simulink model "s_b16a4x1kf"  (R2018a)
settings: Solver=VariableStepDiscrete  StartTime=0.0  StopTime=1000  RelTol=1e-3
undefined symbols (not defined in the file): fft_stages, n_bits_ants, n_bits_xengs
libraries: xbsIndex_r4 x23740, casper_library_misc x48, casper_library_delays x8, xps_library x4, casper_library_scopes x1
(part 89 of 219)

== system s_b16a4x1kf/sys1/xeng/auto_tap/dual_pol_cmac ==
  a1 : Inport
  a2 : Inport  Port=2
  acc_in : Inport  Port=3
  sync : Inport  Port=4
  valid_in : Inport  Port=5
  Concat : xbsIndex_r4/Concat  num_inputs=4  dbl_ovrd=off  block_type=concat
      settings: block_version=9.2.01
  Constant1 : xbsIndex_r4/Constant  const=0  gui_display_data_type=Fixed-point  arith_type=Unsigned  n_bits=1  bin_pt=0  preci_type=Single  exp_width=8  frac_width=24  explicit_period=on  period=1  equ=P=C  opselect=C  inp2=PCIN>>17  opr=+  inp1=P  carry=CIN  dbl_ovrd=off  block_type=constant
      settings: block_version=9.2.01
  Constant2 : xbsIndex_r4/Constant  const=0  gui_display_data_type=Fixed-point  arith_type=Unsigned  n_bits=1  bin_pt=0  preci_type=Single  exp_width=8  frac_width=24  explicit_period=on  period=1  equ=P=C  opselect=C  inp2=PCIN>>17  opr=+  inp1=P  carry=CIN  dbl_ovrd=off  block_type=constant
      settings: block_version=9.2.01
  Constant4 : xbsIndex_r4/Constant  const=0  gui_display_data_type=Fixed-point  arith_type=Unsigned  n_bits=1  bin_pt=0  preci_type=Single  exp_width=8  frac_width=24  explicit_period=on  period=1  equ=P=C  opselect=C  inp2=PCIN>>17  opr=+  inp1=P  carry=CIN  dbl_ovrd=off  block_type=constant
      settings: block_version=9.2.01
  Slice{,1,6,10} (4 alike) : xbsIndex_r4/Slice  nbits=2*n_bits_in  boolean_output=off  mode=Upper Bit Location + Width  bit1=0  base1=MSB of Input  bit0=0  base0=LSB of Input  dbl_ovrd=off  block_type=slice
      settings: block_version=9.2.01
  Slice11 : xbsIndex_r4/Slice  nbits=2*n_bits_out  boolean_output=off  mode=Upper Bit Location + Width  bit1=-6*n_bits_out  base1=MSB of Input  bit0=0  base0=LSB of Input  dbl_ovrd=off  block_type=slice
      settings: infoedit="Extracts a given range of bits from each input sample and presents it at the output.  The output type is ordinarily unsigned with binary point at zero, but can be Boolean when the slice is one bit wide.<P><P>Hardware notes: In hardware this block costs nothing."  block_version=9.2.01
  Slice2 : xbsIndex_r4/Slice  nbits=2*n_bits_out  boolean_output=off  mode=Upper Bit Location + Width  bit1=0  base1=MSB of Input  bit0=0  base0=LSB of Input  dbl_ovrd=off  block_type=slice
      settings: infoedit="Extracts a given range of bits from each input sample and presents it at the output.  The output type is ordinarily unsigned with binary point at zero, but can be Boolean when the slice is one bit wide.<P><P>Hardware notes: In hardware this block costs nothing."  block_version=9.2.01
  Slice{3..4,7,9} (4 alike) : xbsIndex_r4/Slice  nbits=2*n_bits_in  boolean_output=off  mode=Upper Bit Location + Width  bit1=-2*n_bits_in  base1=MSB of Input  bit0=0  base0=LSB of Input  dbl_ovrd=off  block_type=slice
      settings: block_version=9.2.01
  Slice5 : xbsIndex_r4/Slice  nbits=2*n_bits_out  boolean_output=off  mode=Upper Bit Location + Width  bit1=-2*n_bits_out  base1=MSB of Input  bit0=0  base0=LSB of Input  dbl_ovrd=off  block_type=slice
      settings: infoedit="Extracts a given range of bits from each input sample and presents it at the output.  The output type is ordinarily unsigned with binary point at zero, but can be Boolean when the slice is one bit wide.<P><P>Hardware notes: In hardware this block costs nothing."  block_version=9.2.01
  Slice8 : xbsIndex_r4/Slice  nbits=2*n_bits_out  boolean_output=off  mode=Upper Bit Location + Width  bit1=-4*n_bits_out  base1=MSB of Input  bit0=0  base0=LSB of Input  dbl_ovrd=off  block_type=slice
      settings: infoedit="Extracts a given range of bits from each input sample and presents it at the output.  The output type is ordinarily unsigned with binary point at zero, but can be Boolean when the slice is one bit wide.<P><P>Hardware notes: In hardware this block costs nothing."  block_version=9.2.01
  Terminator : Terminator
  Terminator1 : Terminator
  Terminator2 : Terminator
  cmac : Subsystem  Tag=cmac  AncestorBlock=casper_library_correlator/cmac  mask(cmac){acc_len=256, n_bits_a=8, bin_pt_a=7, n_bits_b=8, bin_pt_b=7, quantization=Truncate, overflow=Wrap, mult_latency=4, add_latency=3, in_latency=0, conv_latency=0, multiplier_implementation=embedded multiplier core}
      mask prompts: acc_len "Number of Accumulations"; n_bits_a "Number of bits 'a'"; bin_pt_a "Binary point 'a'"; n_bits_b "Number of bits 'b'"; bin_pt_b "Binary point 'b'"; quantization "Quantisation"; mult_latency "Multiplier Latency"; add_latency "Adder Latency"; in_latency "Input Latency"; conv_latency "Convert Latency"; multiplier_implementation "Multiplier Implementation"
      mask help: A complex multiply-accumulate block. Full precision.
      mask init: same as s_b16a4x1kf/sys0/xeng/auto_tap/dual_pol_cmac/cmac
      mask TypeOptions quantization: Truncate | Round  (unbiased: +/- Inf) | Round  (unbiased: Even Values)
      mask TypeOptions overflow: Wrap | Saturate | Flag as error
      mask TypeOptions multiplier_implementation: behavioral HDL | standard core | embedded multiplier core
  cmac1 : Subsystem  Tag=cmac  AncestorBlock=casper_library_correlator/cmac  mask(cmac){acc_len=256, n_bits_a=8, bin_pt_a=7, n_bits_b=8, bin_pt_b=7, quantization=Truncate, overflow=Wrap, mult_latency=4, add_latency=3, in_latency=0, conv_latency=0, multiplier_implementation=embedded multiplier core}
      mask prompts: acc_len "Number of Accumulations"; n_bits_a "Number of bits 'a'"; bin_pt_a "Binary point 'a'"; n_bits_b "Number of bits 'b'"; bin_pt_b "Binary point 'b'"; quantization "Quantisation"; mult_latency "Multiplier Latency"; add_latency "Adder Latency"; in_latency "Input Latency"; conv_latency "Convert Latency"; multiplier_implementation "Multiplier Implementation"
      mask help: A complex multiply-accumulate block. Full precision.
      mask init: same as s_b16a4x1kf/sys0/xeng/auto_tap/dual_pol_cmac/cmac
      mask TypeOptions quantization: Truncate | Round  (unbiased: +/- Inf) | Round  (unbiased: Even Values)
      mask TypeOptions overflow: Wrap | Saturate | Flag as error
      mask TypeOptions multiplier_implementation: behavioral HDL | standard core | embedded multiplier core
  cmac2 : Subsystem  Tag=cmac  AncestorBlock=casper_library_correlator/cmac  mask(cmac){acc_len=256, n_bits_a=8, bin_pt_a=7, n_bits_b=8, bin_pt_b=7, quantization=Truncate, overflow=Wrap, mult_latency=4, add_latency=3, in_latency=0, conv_latency=0, multiplier_implementation=embedded multiplier core}
      mask prompts: acc_len "Number of Accumulations"; n_bits_a "Number of bits 'a'"; bin_pt_a "Binary point 'a'"; n_bits_b "Number of bits 'b'"; bin_pt_b "Binary point 'b'"; quantization "Quantisation"; mult_latency "Multiplier Latency"; add_latency "Adder Latency"; in_latency "Input Latency"; conv_latency "Convert Latency"; multiplier_implementation "Multiplier Implementation"
      mask help: A complex multiply-accumulate block. Full precision.
      mask init: same as s_b16a4x1kf/sys0/xeng/auto_tap/dual_pol_cmac/cmac
      mask TypeOptions quantization: Truncate | Round  (unbiased: +/- Inf) | Round  (unbiased: Even Values)
      mask TypeOptions overflow: Wrap | Saturate | Flag as error
      mask TypeOptions multiplier_implementation: behavioral HDL | standard core | embedded multiplier core
  cmac3 : Subsystem  Tag=cmac  AncestorBlock=casper_library_correlator/cmac  mask(cmac){acc_len=256, n_bits_a=8, bin_pt_a=7, n_bits_b=8, bin_pt_b=7, quantization=Truncate, overflow=Wrap, mult_latency=4, add_latency=3, in_latency=0, conv_latency=0, multiplier_implementation=embedded multiplier core}
      mask prompts: acc_len "Number of Accumulations"; n_bits_a "Number of bits 'a'"; bin_pt_a "Binary point 'a'"; n_bits_b "Number of bits 'b'"; bin_pt_b "Binary point 'b'"; quantization "Quantisation"; mult_latency "Multiplier Latency"; add_latency "Adder Latency"; in_latency "Input Latency"; conv_latency "Convert Latency"; multiplier_implementation "Multiplier Implementation"
      mask help: A complex multiply-accumulate block. Full precision.
      mask init: same as s_b16a4x1kf/sys0/xeng/auto_tap/dual_pol_cmac/cmac
      mask TypeOptions quantization: Truncate | Round  (unbiased: +/- Inf) | Round  (unbiased: Even Values)
      mask TypeOptions overflow: Wrap | Saturate | Flag as error
      mask TypeOptions multiplier_implementation: behavioral HDL | standard core | embedded multiplier core
  acc_out : Outport
  valid_out : Outport  Port=2
  wires:
  Constant2/1 -> cmac/5(valid_in)
  Slice/1 -> cmac/1(a+bi)
  Slice1/1 -> cmac/2(c+di)
  Slice2/1 -> cmac/3(acc_in)
  Slice3/1 -> cmac1/1(a+bi)
  Slice4/1 -> cmac1/2(c+di)
  Slice5/1 -> cmac1/3(acc_in)
  Concat/1 -> acc_out/1
  valid_in/1 -> cmac3/5(valid_in)
  cmac/2(valid_out) -> Terminator/1
  Constant1/1 -> cmac1/5(valid_in)
  Slice6/1 -> cmac2/1(a+bi)
  Slice7/1 -> cmac2/2(c+di)
  Slice8/1 -> cmac2/3(acc_in)
  Constant4/1 -> cmac2/5(valid_in)
  Slice9/1 -> cmac3/1(a+bi)
  Slice10/1 -> cmac3/2(c+di)
  Slice11/1 -> cmac3/3(acc_in)
  sync/1 -> cmac/4(sync), cmac1/4(sync), cmac2/4(sync), cmac3/4(sync)
  cmac1/2(valid_out) -> Terminator1/1
  cmac2/2(valid_out) -> Terminator2/1
  cmac3/2(valid_out) -> valid_out/1
  cmac/1(acc_out) -> Concat/1
  cmac1/1(acc_out) -> Concat/2
  cmac2/1(acc_out) -> Concat/3
  cmac3/1(acc_out) -> Concat/4
  a1/1 -> Slice/1, Slice3/1, Slice6/1, Slice9/1
  a2/1 -> Slice1/1, Slice4/1, Slice7/1, Slice10/1
  acc_in/1 -> Slice11/1, Slice8/1, Slice5/1, Slice2/1

== system s_b16a4x1kf/sys1/xeng/baseline_tap1/delay ==
  din : Inport
  constant : xbsIndex_r4/Constant  const=1  gui_display_data_type=Fixed-point  arith_type=Boolean  n_bits=16  bin_pt=14  preci_type=Single  exp_width=8  frac_width=24  explicit_period=on  period=1  equ=P=C  opselect=C  inp2=PCIN>>17  opr=+  inp1=P  carry=CIN  dbl_ovrd=off  block_type=constant
  counter : xbsIndex_r4/Counter  cnt_type=Count Limited  cnt_to=DelayLen - bram_latency - 1  operation=Up  start_count=0  cnt_by_val=1  arith_type=Unsigned  n_bits=8  bin_pt=0  load_pin=off  rst=off  en=off  explicit_period=on  period=1  use_behavioral_HDL=on  implementation=Fabric  use_rpm=off  dbl_ovrd=off  block_type=counter
  d{1..6} (6 alike) : xbsIndex_r4/Delay  rst=off  infoeditControl=Selection of Reset will increase slice count due to use of real FFs and instead of SRLs  en=off  latency=1  reg_retiming=on  dbl_ovrd=off  block_type=delay
  ram : xbsIndex_r4/Single Port RAM  depth=256  initVector=0  distributed_mem=Block RAM  write_mode=Read Before Write  rst=off  init_reg=0  en=off  latency=1  optimize=Area  dbl_ovrd=off  block_type=spram
  dout : Outport
  wires:
  counter/1 -> ram/1
  din/1 -> ram/2
  constant/1 -> ram/3
  ram/1 -> d1/1
  d1/1 -> d2/1
  d2/1 -> d3/1
  d3/1 -> d4/1
  d4/1 -> d5/1
  d5/1 -> d6/1
  d6/1 -> dout/1

== system s_b16a4x1kf/sys1/xeng/baseline_tap1/dual_pol_cmac ==
  a1 : Inport
  a2 : Inport  Port=2
  acc_in : Inport  Port=3
  sync : Inport  Port=4
  valid_in : Inport  Port=5
  Concat : xbsIndex_r4/Concat  num_inputs=4  dbl_ovrd=off  block_type=concat
      settings: block_version=9.2.01
  Constant1 : xbsIndex_r4/Constant  const=0  gui_display_data_type=Fixed-point  arith_type=Unsigned  n_bits=1  bin_pt=0  preci_type=Single  exp_width=8  frac_width=24  explicit_period=on  period=1  equ=P=C  opselect=C  inp2=PCIN>>17  opr=+  inp1=P  carry=CIN  dbl_ovrd=off  block_type=constant
      settings: block_version=9.2.01
  Constant2 : xbsIndex_r4/Constant  const=0  gui_display_data_type=Fixed-point  arith_type=Unsigned  n_bits=1  bin_pt=0  preci_type=Single  exp_width=8  frac_width=24  explicit_period=on  period=1  equ=P=C  opselect=C  inp2=PCIN>>17  opr=+  inp1=P  carry=CIN  dbl_ovrd=off  block_type=constant
      settings: block_version=9.2.01
  Constant4 : xbsIndex_r4/Constant  const=0  gui_display_data_type=Fixed-point  arith_type=Unsigned  n_bits=1  bin_pt=0  preci_type=Single  exp_width=8  frac_width=24  explicit_period=on  period=1  equ=P=C  opselect=C  inp2=PCIN>>17  opr=+  inp1=P  carry=CIN  dbl_ovrd=off  block_type=constant
      settings: block_version=9.2.01
  Slice{,1,6,10} (4 alike) : xbsIndex_r4/Slice  nbits=2*n_bits_in  boolean_output=off  mode=Upper Bit Location + Width  bit1=0  base1=MSB of Input  bit0=0  base0=LSB of Input  dbl_ovrd=off  block_type=slice
      settings: block_version=9.2.01
  Slice11 : xbsIndex_r4/Slice  nbits=2*n_bits_out  boolean_output=off  mode=Upper Bit Location + Width  bit1=-6*n_bits_out  base1=MSB of Input  bit0=0  base0=LSB of Input  dbl_ovrd=off  block_type=slice
      settings: infoedit="Extracts a given range of bits from each input sample and presents it at the output.  The output type is ordinarily unsigned with binary point at zero, but can be Boolean when the slice is one bit wide.<P><P>Hardware notes: In hardware this block costs nothing."  block_version=9.2.01
  Slice2 : xbsIndex_r4/Slice  nbits=2*n_bits_out  boolean_output=off  mode=Upper Bit Location + Width  bit1=0  base1=MSB of Input  bit0=0  base0=LSB of Input  dbl_ovrd=off  block_type=slice
      settings: infoedit="Extracts a given range of bits from each input sample and presents it at the output.  The output type is ordinarily unsigned with binary point at zero, but can be Boolean when the slice is one bit wide.<P><P>Hardware notes: In hardware this block costs nothing."  block_version=9.2.01
  Slice{3..4,7,9} (4 alike) : xbsIndex_r4/Slice  nbits=2*n_bits_in  boolean_output=off  mode=Upper Bit Location + Width  bit1=-2*n_bits_in  base1=MSB of Input  bit0=0  base0=LSB of Input  dbl_ovrd=off  block_type=slice
      settings: block_version=9.2.01
  Slice5 : xbsIndex_r4/Slice  nbits=2*n_bits_out  boolean_output=off  mode=Upper Bit Location + Width  bit1=-2*n_bits_out  base1=MSB of Input  bit0=0  base0=LSB of Input  dbl_ovrd=off  block_type=slice
      settings: infoedit="Extracts a given range of bits from each input sample and presents it at the output.  The output type is ordinarily unsigned with binary point at zero, but can be Boolean when the slice is one bit wide.<P><P>Hardware notes: In hardware this block costs nothing."  block_version=9.2.01
  Slice8 : xbsIndex_r4/Slice  nbits=2*n_bits_out  boolean_output=off  mode=Upper Bit Location + Width  bit1=-4*n_bits_out  base1=MSB of Input  bit0=0  base0=LSB of Input  dbl_ovrd=off  block_type=slice
      settings: infoedit="Extracts a given range of bits from each input sample and presents it at the output.  The output type is ordinarily unsigned with binary point at zero, but can be Boolean when the slice is one bit wide.<P><P>Hardware notes: In hardware this block costs nothing."  block_version=9.2.01
  Terminator : Terminator
  Terminator1 : Terminator
  Terminator2 : Terminator
  cmac : Subsystem  Tag=cmac  AncestorBlock=casper_library_correlator/cmac  mask(cmac){acc_len=256, n_bits_a=8, bin_pt_a=7, n_bits_b=8, bin_pt_b=7, quantization=Truncate, overflow=Wrap, mult_latency=4, add_latency=3, in_latency=0, conv_latency=0, multiplier_implementation=embedded multiplier core}
      mask prompts: acc_len "Number of Accumulations"; n_bits_a "Number of bits 'a'"; bin_pt_a "Binary point 'a'"; n_bits_b "Number of bits 'b'"; bin_pt_b "Binary point 'b'"; quantization "Quantisation"; mult_latency "Multiplier Latency"; add_latency "Adder Latency"; in_latency "Input Latency"; conv_latency "Convert Latency"; multiplier_implementation "Multiplier Implementation"
      mask help: A complex multiply-accumulate block. Full precision.
      mask init: same as s_b16a4x1kf/sys0/xeng/auto_tap/dual_pol_cmac/cmac
      mask TypeOptions quantization: Truncate | Round  (unbiased: +/- Inf) | Round  (unbiased: Even Values)
      mask TypeOptions overflow: Wrap | Saturate | Flag as error
      mask TypeOptions multiplier_implementation: behavioral HDL | standard core | embedded multiplier core
  cmac1 : Subsystem  Tag=cmac  AncestorBlock=casper_library_correlator/cmac  mask(cmac){acc_len=256, n_bits_a=8, bin_pt_a=7, n_bits_b=8, bin_pt_b=7, quantization=Truncate, overflow=Wrap, mult_latency=4, add_latency=3, in_latency=0, conv_latency=0, multiplier_implementation=embedded multiplier core}
      mask prompts: acc_len "Number of Accumulations"; n_bits_a "Number of bits 'a'"; bin_pt_a "Binary point 'a'"; n_bits_b "Number of bits 'b'"; bin_pt_b "Binary point 'b'"; quantization "Quantisation"; mult_latency "Multiplier Latency"; add_latency "Adder Latency"; in_latency "Input Latency"; conv_latency "Convert Latency"; multiplier_implementation "Multiplier Implementation"
      mask help: A complex multiply-accumulate block. Full precision.
      mask init: same as s_b16a4x1kf/sys0/xeng/auto_tap/dual_pol_cmac/cmac
      mask TypeOptions quantization: Truncate | Round  (unbiased: +/- Inf) | Round  (unbiased: Even Values)
      mask TypeOptions overflow: Wrap | Saturate | Flag as error
      mask TypeOptions multiplier_implementation: behavioral HDL | standard core | embedded multiplier core
  cmac2 : Subsystem  Tag=cmac  AncestorBlock=casper_library_correlator/cmac  mask(cmac){acc_len=256, n_bits_a=8, bin_pt_a=7, n_bits_b=8, bin_pt_b=7, quantization=Truncate, overflow=Wrap, mult_latency=4, add_latency=3, in_latency=0, conv_latency=0, multiplier_implementation=embedded multiplier core}
      mask prompts: acc_len "Number of Accumulations"; n_bits_a "Number of bits 'a'"; bin_pt_a "Binary point 'a'"; n_bits_b "Number of bits 'b'"; bin_pt_b "Binary point 'b'"; quantization "Quantisation"; mult_latency "Multiplier Latency"; add_latency "Adder Latency"; in_latency "Input Latency"; conv_latency "Convert Latency"; multiplier_implementation "Multiplier Implementation"
      mask help: A complex multiply-accumulate block. Full precision.
      mask init: same as s_b16a4x1kf/sys0/xeng/auto_tap/dual_pol_cmac/cmac
      mask TypeOptions quantization: Truncate | Round  (unbiased: +/- Inf) | Round  (unbiased: Even Values)
      mask TypeOptions overflow: Wrap | Saturate | Flag as error
      mask TypeOptions multiplier_implementation: behavioral HDL | standard core | embedded multiplier core
  cmac3 : Subsystem  Tag=cmac  AncestorBlock=casper_library_correlator/cmac  mask(cmac){acc_len=256, n_bits_a=8, bin_pt_a=7, n_bits_b=8, bin_pt_b=7, quantization=Truncate, overflow=Wrap, mult_latency=4, add_latency=3, in_latency=0, conv_latency=0, multiplier_implementation=embedded multiplier core}
      mask prompts: acc_len "Number of Accumulations"; n_bits_a "Number of bits 'a'"; bin_pt_a "Binary point 'a'"; n_bits_b "Number of bits 'b'"; bin_pt_b "Binary point 'b'"; quantization "Quantisation"; mult_latency "Multiplier Latency"; add_latency "Adder Latency"; in_latency "Input Latency"; conv_latency "Convert Latency"; multiplier_implementation "Multiplier Implementation"
      mask help: A complex multiply-accumulate block. Full precision.
      mask init: same as s_b16a4x1kf/sys0/xeng/auto_tap/dual_pol_cmac/cmac
      mask TypeOptions quantization: Truncate | Round  (unbiased: +/- Inf) | Round  (unbiased: Even Values)
      mask TypeOptions overflow: Wrap | Saturate | Flag as error
      mask TypeOptions multiplier_implementation: behavioral HDL | standard core | embedded multiplier core
  acc_out : Outport
  valid_out : Outport  Port=2
  wires:
  Constant2/1 -> cmac/5(valid_in)
  Slice/1 -> cmac/1(a+bi)
  Slice1/1 -> cmac/2(c+di)
  Slice2/1 -> cmac/3(acc_in)
  Slice3/1 -> cmac1/1(a+bi)
  Slice4/1 -> cmac1/2(c+di)
  Slice5/1 -> cmac1/3(acc_in)
  Concat/1 -> acc_out/1
  valid_in/1 -> cmac3/5(valid_in)
  cmac/2(valid_out) -> Terminator/1
  Constant1/1 -> cmac1/5(valid_in)
  Slice6/1 -> cmac2/1(a+bi)
  Slice7/1 -> cmac2/2(c+di)
  Slice8/1 -> cmac2/3(acc_in)
  Constant4/1 -> cmac2/5(valid_in)
  Slice9/1 -> cmac3/1(a+bi)
  Slice10/1 -> cmac3/2(c+di)
  Slice11/1 -> cmac3/3(acc_in)
  sync/1 -> cmac/4(sync), cmac1/4(sync), cmac2/4(sync), cmac3/4(sync)
  cmac1/2(valid_out) -> Terminator1/1
  cmac2/2(valid_out) -> Terminator2/1
  cmac3/2(valid_out) -> valid_out/1
  cmac/1(acc_out) -> Concat/1
  cmac1/1(acc_out) -> Concat/2
  cmac2/1(acc_out) -> Concat/3
  cmac3/1(acc_out) -> Concat/4
  a1/1 -> Slice/1, Slice3/1, Slice6/1, Slice9/1
  a2/1 -> Slice1/1, Slice4/1, Slice7/1, Slice10/1
  acc_in/1 -> Slice11/1, Slice8/1, Slice5/1, Slice2/1

== system s_b16a4x1kf/sys1/xeng/baseline_tap2/delay ==
  din : Inport
  constant : xbsIndex_r4/Constant  const=1  gui_display_data_type=Fixed-point  arith_type=Boolean  n_bits=16  bin_pt=14  preci_type=Single  exp_width=8  frac_width=24  explicit_period=on  period=1  equ=P=C  opselect=C  inp2=PCIN>>17  opr=+  inp1=P  carry=CIN  dbl_ovrd=off  block_type=constant
  counter : xbsIndex_r4/Counter  cnt_type=Count Limited  cnt_to=DelayLen - bram_latency - 1  operation=Up  start_count=0  cnt_by_val=1  arith_type=Unsigned  n_bits=8  bin_pt=0  load_pin=off  rst=off  en=off  explicit_period=on  period=1  use_behavioral_HDL=on  implementation=Fabric  use_rpm=off  dbl_ovrd=off  block_type=counter
  d{1..6} (6 alike) : xbsIndex_r4/Delay  rst=off  infoeditControl=Selection of Reset will increase slice count due to use of real FFs and instead of SRLs  en=off  latency=1  reg_retiming=on  dbl_ovrd=off  block_type=delay
  ram : xbsIndex_r4/Single Port RAM  depth=256  initVector=0  distributed_mem=Block RAM  write_mode=Read Before Write  rst=off  init_reg=0  en=off  latency=1  optimize=Area  dbl_ovrd=off  block_type=spram
  dout : Outport
  wires:
  counter/1 -> ram/1
  din/1 -> ram/2
  constant/1 -> ram/3
  ram/1 -> d1/1
  d1/1 -> d2/1
  d2/1 -> d3/1
  d3/1 -> d4/1
  d4/1 -> d5/1
  d5/1 -> d6/1
  d6/1 -> dout/1

== system s_b16a4x1kf/sys1/xeng/baseline_tap2/dual_pol_cmac ==
  a1 : Inport
  a2 : Inport  Port=2
  acc_in : Inport  Port=3
  sync : Inport  Port=4
  valid_in : Inport  Port=5
  Concat : xbsIndex_r4/Concat  num_inputs=4  dbl_ovrd=off  block_type=concat
      settings: block_version=9.2.01
  Constant1 : xbsIndex_r4/Constant  const=0  gui_display_data_type=Fixed-point  arith_type=Unsigned  n_bits=1  bin_pt=0  preci_type=Single  exp_width=8  frac_width=24  explicit_period=on  period=1  equ=P=C  opselect=C  inp2=PCIN>>17  opr=+  inp1=P  carry=CIN  dbl_ovrd=off  block_type=constant
      settings: block_version=9.2.01
  Constant2 : xbsIndex_r4/Constant  const=0  gui_display_data_type=Fixed-point  arith_type=Unsigned  n_bits=1  bin_pt=0  preci_type=Single  exp_width=8  frac_width=24  explicit_period=on  period=1  equ=P=C  opselect=C  inp2=PCIN>>17  opr=+  inp1=P  carry=CIN  dbl_ovrd=off  block_type=constant
      settings: block_version=9.2.01
  Constant4 : xbsIndex_r4/Constant  const=0  gui_display_data_type=Fixed-point  arith_type=Unsigned  n_bits=1  bin_pt=0  preci_type=Single  exp_width=8  frac_width=24  explicit_period=on  period=1  equ=P=C  opselect=C  inp2=PCIN>>17  opr=+  inp1=P  carry=CIN  dbl_ovrd=off  block_type=constant
      settings: block_version=9.2.01
  Slice{,1,6,10} (4 alike) : xbsIndex_r4/Slice  nbits=2*n_bits_in  boolean_output=off  mode=Upper Bit Location + Width  bit1=0  base1=MSB of Input  bit0=0  base0=LSB of Input  dbl_ovrd=off  block_type=slice
      settings: block_version=9.2.01
  Slice11 : xbsIndex_r4/Slice  nbits=2*n_bits_out  boolean_output=off  mode=Upper Bit Location + Width  bit1=-6*n_bits_out  base1=MSB of Input  bit0=0  base0=LSB of Input  dbl_ovrd=off  block_type=slice
      settings: infoedit="Extracts a given range of bits from each input sample and presents it at the output.  The output type is ordinarily unsigned with binary point at zero, but can be Boolean when the slice is one bit wide.<P><P>Hardware notes: In hardware this block costs nothing."  block_version=9.2.01
  Slice2 : xbsIndex_r4/Slice  nbits=2*n_bits_out  boolean_output=off  mode=Upper Bit Location + Width  bit1=0  base1=MSB of Input  bit0=0  base0=LSB of Input  dbl_ovrd=off  block_type=slice
      settings: infoedit="Extracts a given range of bits from each input sample and presents it at the output.  The output type is ordinarily unsigned with binary point at zero, but can be Boolean when the slice is one bit wide.<P><P>Hardware notes: In hardware this block costs nothing."  block_version=9.2.01
  Slice{3..4,7,9} (4 alike) : xbsIndex_r4/Slice  nbits=2*n_bits_in  boolean_output=off  mode=Upper Bit Location + Width  bit1=-2*n_bits_in  base1=MSB of Input  bit0=0  base0=LSB of Input  dbl_ovrd=off  block_type=slice
      settings: block_version=9.2.01
  Slice5 : xbsIndex_r4/Slice  nbits=2*n_bits_out  boolean_output=off  mode=Upper Bit Location + Width  bit1=-2*n_bits_out  base1=MSB of Input  bit0=0  base0=LSB of Input  dbl_ovrd=off  block_type=slice
      settings: infoedit="Extracts a given range of bits from each input sample and presents it at the output.  The output type is ordinarily unsigned with binary point at zero, but can be Boolean when the slice is one bit wide.<P><P>Hardware notes: In hardware this block costs nothing."  block_version=9.2.01
  Slice8 : xbsIndex_r4/Slice  nbits=2*n_bits_out  boolean_output=off  mode=Upper Bit Location + Width  bit1=-4*n_bits_out  base1=MSB of Input  bit0=0  base0=LSB of Input  dbl_ovrd=off  block_type=slice
      settings: infoedit="Extracts a given range of bits from each input sample and presents it at the output.  The output type is ordinarily unsigned with binary point at zero, but can be Boolean when the slice is one bit wide.<P><P>Hardware notes: In hardware this block costs nothing."  block_version=9.2.01
  Terminator : Terminator
  Terminator1 : Terminator
  Terminator2 : Terminator
  cmac : Subsystem  Tag=cmac  AncestorBlock=casper_library_correlator/cmac  mask(cmac){acc_len=256, n_bits_a=8, bin_pt_a=7, n_bits_b=8, bin_pt_b=7, quantization=Truncate, overflow=Wrap, mult_latency=4, add_latency=3, in_latency=0, conv_latency=0, multiplier_implementation=embedded multiplier core}
      mask prompts: acc_len "Number of Accumulations"; n_bits_a "Number of bits 'a'"; bin_pt_a "Binary point 'a'"; n_bits_b "Number of bits 'b'"; bin_pt_b "Binary point 'b'"; quantization "Quantisation"; mult_latency "Multiplier Latency"; add_latency "Adder Latency"; in_latency "Input Latency"; conv_latency "Convert Latency"; multiplier_implementation "Multiplier Implementation"
      mask help: A complex multiply-accumulate block. Full precision.
      mask init: same as s_b16a4x1kf/sys0/xeng/auto_tap/dual_pol_cmac/cmac
      mask TypeOptions quantization: Truncate | Round  (unbiased: +/- Inf) | Round  (unbiased: Even Values)
      mask TypeOptions overflow: Wrap | Saturate | Flag as error
      mask TypeOptions multiplier_implementation: behavioral HDL | standard core | embedded multiplier core
  cmac1 : Subsystem  Tag=cmac  AncestorBlock=casper_library_correlator/cmac  mask(cmac){acc_len=256, n_bits_a=8, bin_pt_a=7, n_bits_b=8, bin_pt_b=7, quantization=Truncate, overflow=Wrap, mult_latency=4, add_latency=3, in_latency=0, conv_latency=0, multiplier_implementation=embedded multiplier core}
      mask prompts: acc_len "Number of Accumulations"; n_bits_a "Number of bits 'a'"; bin_pt_a "Binary point 'a'"; n_bits_b "Number of bits 'b'"; bin_pt_b "Binary point 'b'"; quantization "Quantisation"; mult_latency "Multiplier Latency"; add_latency "Adder Latency"; in_latency "Input Latency"; conv_latency "Convert Latency"; multiplier_implementation "Multiplier Implementation"
      mask help: A complex multiply-accumulate block. Full precision.
      mask init: same as s_b16a4x1kf/sys0/xeng/auto_tap/dual_pol_cmac/cmac
      mask TypeOptions quantization: Truncate | Round  (unbiased: +/- Inf) | Round  (unbiased: Even Values)
      mask TypeOptions overflow: Wrap | Saturate | Flag as error
      mask TypeOptions multiplier_implementation: behavioral HDL | standard core | embedded multiplier core
  cmac2 : Subsystem  Tag=cmac  AncestorBlock=casper_library_correlator/cmac  mask(cmac){acc_len=256, n_bits_a=8, bin_pt_a=7, n_bits_b=8, bin_pt_b=7, quantization=Truncate, overflow=Wrap, mult_latency=4, add_latency=3, in_latency=0, conv_latency=0, multiplier_implementation=embedded multiplier core}
      mask prompts: acc_len "Number of Accumulations"; n_bits_a "Number of bits 'a'"; bin_pt_a "Binary point 'a'"; n_bits_b "Number of bits 'b'"; bin_pt_b "Binary point 'b'"; quantization "Quantisation"; mult_latency "Multiplier Latency"; add_latency "Adder Latency"; in_latency "Input Latency"; conv_latency "Convert Latency"; multiplier_implementation "Multiplier Implementation"
      mask help: A complex multiply-accumulate block. Full precision.
      mask init: same as s_b16a4x1kf/sys0/xeng/auto_tap/dual_pol_cmac/cmac
      mask TypeOptions quantization: Truncate | Round  (unbiased: +/- Inf) | Round  (unbiased: Even Values)
      mask TypeOptions overflow: Wrap | Saturate | Flag as error
      mask TypeOptions multiplier_implementation: behavioral HDL | standard core | embedded multiplier core
  cmac3 : Subsystem  Tag=cmac  AncestorBlock=casper_library_correlator/cmac  mask(cmac){acc_len=256, n_bits_a=8, bin_pt_a=7, n_bits_b=8, bin_pt_b=7, quantization=Truncate, overflow=Wrap, mult_latency=4, add_latency=3, in_latency=0, conv_latency=0, multiplier_implementation=embedded multiplier core}
      mask prompts: acc_len "Number of Accumulations"; n_bits_a "Number of bits 'a'"; bin_pt_a "Binary point 'a'"; n_bits_b "Number of bits 'b'"; bin_pt_b "Binary point 'b'"; quantization "Quantisation"; mult_latency "Multiplier Latency"; add_latency "Adder Latency"; in_latency "Input Latency"; conv_latency "Convert Latency"; multiplier_implementation "Multiplier Implementation"
      mask help: A complex multiply-accumulate block. Full precision.
      mask init: same as s_b16a4x1kf/sys0/xeng/auto_tap/dual_pol_cmac/cmac
      mask TypeOptions quantization: Truncate | Round  (unbiased: +/- Inf) | Round  (unbiased: Even Values)
      mask TypeOptions overflow: Wrap | Saturate | Flag as error
      mask TypeOptions multiplier_implementation: behavioral HDL | standard core | embedded multiplier core
  acc_out : Outport
  valid_out : Outport  Port=2
  wires:
  Constant2/1 -> cmac/5(valid_in)
  Slice/1 -> cmac/1(a+bi)
  Slice1/1 -> cmac/2(c+di)
  Slice2/1 -> cmac/3(acc_in)
  Slice3/1 -> cmac1/1(a+bi)
  Slice4/1 -> cmac1/2(c+di)
  Slice5/1 -> cmac1/3(acc_in)
  Concat/1 -> acc_out/1
  valid_in/1 -> cmac3/5(valid_in)
  cmac/2(valid_out) -> Terminator/1
  Constant1/1 -> cmac1/5(valid_in)
  Slice6/1 -> cmac2/1(a+bi)
  Slice7/1 -> cmac2/2(c+di)
  Slice8/1 -> cmac2/3(acc_in)
  Constant4/1 -> cmac2/5(valid_in)
  Slice9/1 -> cmac3/1(a+bi)
  Slice10/1 -> cmac3/2(c+di)
  Slice11/1 -> cmac3/3(acc_in)
  sync/1 -> cmac/4(sync), cmac1/4(sync), cmac2/4(sync), cmac3/4(sync)
  cmac1/2(valid_out) -> Terminator1/1
  cmac2/2(valid_out) -> Terminator2/1
  cmac3/2(valid_out) -> valid_out/1
  cmac/1(acc_out) -> Concat/1
  cmac1/1(acc_out) -> Concat/2
  cmac2/1(acc_out) -> Concat/3
  cmac3/1(acc_out) -> Concat/4
  a1/1 -> Slice/1, Slice3/1, Slice6/1, Slice9/1
  a2/1 -> Slice1/1, Slice4/1, Slice7/1, Slice10/1
  acc_in/1 -> Slice11/1, Slice8/1, Slice5/1, Slice2/1

== system s_b16a4x1kf/sys1/xeng/baseline_tap3/delay ==
  din : Inport
  constant : xbsIndex_r4/Constant  const=1  gui_display_data_type=Fixed-point  arith_type=Boolean  n_bits=16  bin_pt=14  preci_type=Single  exp_width=8  frac_width=24  explicit_period=on  period=1  equ=P=C  opselect=C  inp2=PCIN>>17  opr=+  inp1=P  carry=CIN  dbl_ovrd=off  block_type=constant
  counter : xbsIndex_r4/Counter  cnt_type=Count Limited  cnt_to=DelayLen - bram_latency - 1  operation=Up  start_count=0  cnt_by_val=1  arith_type=Unsigned  n_bits=8  bin_pt=0  load_pin=off  rst=off  en=off  explicit_period=on  period=1  use_behavioral_HDL=on  implementation=Fabric  use_rpm=off  dbl_ovrd=off  block_type=counter
  d{1..6} (6 alike) : xbsIndex_r4/Delay  rst=off  infoeditControl=Selection of Reset will increase slice count due to use of real FFs and instead of SRLs  en=off  latency=1  reg_retiming=on  dbl_ovrd=off  block_type=delay
  ram : xbsIndex_r4/Single Port RAM  depth=256  initVector=0  distributed_mem=Block RAM  write_mode=Read Before Write  rst=off  init_reg=0  en=off  latency=1  optimize=Area  dbl_ovrd=off  block_type=spram
  dout : Outport
  wires:
  counter/1 -> ram/1
  din/1 -> ram/2
  constant/1 -> ram/3
  ram/1 -> d1/1
  d1/1 -> d2/1
  d2/1 -> d3/1
  d3/1 -> d4/1
  d4/1 -> d5/1
  d5/1 -> d6/1
  d6/1 -> dout/1

== system s_b16a4x1kf/sys1/xeng/baseline_tap3/dual_pol_cmac ==
  a1 : Inport
  a2 : Inport  Port=2
  acc_in : Inport  Port=3
  sync : Inport  Port=4
  valid_in : Inport  Port=5
  Concat : xbsIndex_r4/Concat  num_inputs=4  dbl_ovrd=off  block_type=concat
      settings: block_version=9.2.01
  Constant1 : xbsIndex_r4/Constant  const=0  gui_display_data_type=Fixed-point  arith_type=Unsigned  n_bits=1  bin_pt=0  preci_type=Single  exp_width=8  frac_width=24  explicit_period=on  period=1  equ=P=C  opselect=C  inp2=PCIN>>17  opr=+  inp1=P  carry=CIN  dbl_ovrd=off  block_type=constant
      settings: block_version=9.2.01
  Constant2 : xbsIndex_r4/Constant  const=0  gui_display_data_type=Fixed-point  arith_type=Unsigned  n_bits=1  bin_pt=0  preci_type=Single  exp_width=8  frac_width=24  explicit_period=on  period=1  equ=P=C  opselect=C  inp2=PCIN>>17  opr=+  inp1=P  carry=CIN  dbl_ovrd=off  block_type=constant
      settings: block_version=9.2.01
  Constant4 : xbsIndex_r4/Constant  const=0  gui_display_data_type=Fixed-point  arith_type=Unsigned  n_bits=1  bin_pt=0  preci_type=Single  exp_width=8  frac_width=24  explicit_period=on  period=1  equ=P=C  opselect=C  inp2=PCIN>>17  opr=+  inp1=P  carry=CIN  dbl_ovrd=off  block_type=constant
      settings: block_version=9.2.01
  Slice{,1,6,10} (4 alike) : xbsIndex_r4/Slice  nbits=2*n_bits_in  boolean_output=off  mode=Upper Bit Location + Width  bit1=0  base1=MSB of Input  bit0=0  base0=LSB of Input  dbl_ovrd=off  block_type=slice
      settings: block_version=9.2.01
  Slice11 : xbsIndex_r4/Slice  nbits=2*n_bits_out  boolean_output=off  mode=Upper Bit Location + Width  bit1=-6*n_bits_out  base1=MSB of Input  bit0=0  base0=LSB of Input  dbl_ovrd=off  block_type=slice
      settings: infoedit="Extracts a given range of bits from each input sample and presents it at the output.  The output type is ordinarily unsigned with binary point at zero, but can be Boolean when the slice is one bit wide.<P><P>Hardware notes: In hardware this block costs nothing."  block_version=9.2.01
  Slice2 : xbsIndex_r4/Slice  nbits=2*n_bits_out  boolean_output=off  mode=Upper Bit Location + Width  bit1=0  base1=MSB of Input  bit0=0  base0=LSB of Input  dbl_ovrd=off  block_type=slice
      settings: infoedit="Extracts a given range of bits from each input sample and presents it at the output.  The output type is ordinarily unsigned with binary point at zero, but can be Boolean when the slice is one bit wide.<P><P>Hardware notes: In hardware this block costs nothing."  block_version=9.2.01
  Slice{3..4,7,9} (4 alike) : xbsIndex_r4/Slice  nbits=2*n_bits_in  boolean_output=off  mode=Upper Bit Location + Width  bit1=-2*n_bits_in  base1=MSB of Input  bit0=0  base0=LSB of Input  dbl_ovrd=off  block_type=slice
      settings: block_version=9.2.01
  Slice5 : xbsIndex_r4/Slice  nbits=2*n_bits_out  boolean_output=off  mode=Upper Bit Location + Width  bit1=-2*n_bits_out  base1=MSB of Input  bit0=0  base0=LSB of Input  dbl_ovrd=off  block_type=slice
      settings: infoedit="Extracts a given range of bits from each input sample and presents it at the output.  The output type is ordinarily unsigned with binary point at zero, but can be Boolean when the slice is one bit wide.<P><P>Hardware notes: In hardware this block costs nothing."  block_version=9.2.01
  Slice8 : xbsIndex_r4/Slice  nbits=2*n_bits_out  boolean_output=off  mode=Upper Bit Location + Width  bit1=-4*n_bits_out  base1=MSB of Input  bit0=0  base0=LSB of Input  dbl_ovrd=off  block_type=slice
      settings: infoedit="Extracts a given range of bits from each input sample and presents it at the output.  The output type is ordinarily unsigned with binary point at zero, but can be Boolean when the slice is one bit wide.<P><P>Hardware notes: In hardware this block costs nothing."  block_version=9.2.01
  Terminator : Terminator
  Terminator1 : Terminator
  Terminator2 : Terminator
  cmac : Subsystem  Tag=cmac  AncestorBlock=casper_library_correlator/cmac  mask(cmac){acc_len=256, n_bits_a=8, bin_pt_a=7, n_bits_b=8, bin_pt_b=7, quantization=Truncate, overflow=Wrap, mult_latency=4, add_latency=3, in_latency=0, conv_latency=0, multiplier_implementation=embedded multiplier core}
      mask prompts: acc_len "Number of Accumulations"; n_bits_a "Number of bits 'a'"; bin_pt_a "Binary point 'a'"; n_bits_b "Number of bits 'b'"; bin_pt_b "Binary point 'b'"; quantization "Quantisation"; mult_latency "Multiplier Latency"; add_latency "Adder Latency"; in_latency "Input Latency"; conv_latency "Convert Latency"; multiplier_implementation "Multiplier Implementation"
      mask help: A complex multiply-accumulate block. Full precision.
      mask init: same as s_b16a4x1kf/sys0/xeng/auto_tap/dual_pol_cmac/cmac
      mask TypeOptions quantization: Truncate | Round  (unbiased: +/- Inf) | Round  (unbiased: Even Values)
      mask TypeOptions overflow: Wrap | Saturate | Flag as error
      mask TypeOptions multiplier_implementation: behavioral HDL | standard core | embedded multiplier core
  cmac1 : Subsystem  Tag=cmac  AncestorBlock=casper_library_correlator/cmac  mask(cmac){acc_len=256, n_bits_a=8, bin_pt_a=7, n_bits_b=8, bin_pt_b=7, quantization=Truncate, overflow=Wrap, mult_latency=4, add_latency=3, in_latency=0, conv_latency=0, multiplier_implementation=embedded multiplier core}
      mask prompts: acc_len "Number of Accumulations"; n_bits_a "Number of bits 'a'"; bin_pt_a "Binary point 'a'"; n_bits_b "Number of bits 'b'"; bin_pt_b "Binary point 'b'"; quantization "Quantisation"; mult_latency "Multiplier Latency"; add_latency "Adder Latency"; in_latency "Input Latency"; conv_latency "Convert Latency"; multiplier_implementation "Multiplier Implementation"
      mask help: A complex multiply-accumulate block. Full precision.
      mask init: same as s_b16a4x1kf/sys0/xeng/auto_tap/dual_pol_cmac/cmac
      mask TypeOptions quantization: Truncate | Round  (unbiased: +/- Inf) | Round  (unbiased: Even Values)
      mask TypeOptions overflow: Wrap | Saturate | Flag as error
      mask TypeOptions multiplier_implementation: behavioral HDL | standard core | embedded multiplier core
  cmac2 : Subsystem  Tag=cmac  AncestorBlock=casper_library_correlator/cmac  mask(cmac){acc_len=256, n_bits_a=8, bin_pt_a=7, n_bits_b=8, bin_pt_b=7, quantization=Truncate, overflow=Wrap, mult_latency=4, add_latency=3, in_latency=0, conv_latency=0, multiplier_implementation=embedded multiplier core}
      mask prompts: acc_len "Number of Accumulations"; n_bits_a "Number of bits 'a'"; bin_pt_a "Binary point 'a'"; n_bits_b "Number of bits 'b'"; bin_pt_b "Binary point 'b'"; quantization "Quantisation"; mult_latency "Multiplier Latency"; add_latency "Adder Latency"; in_latency "Input Latency"; conv_latency "Convert Latency"; multiplier_implementation "Multiplier Implementation"
      mask help: A complex multiply-accumulate block. Full precision.
      mask init: same as s_b16a4x1kf/sys0/xeng/auto_tap/dual_pol_cmac/cmac
      mask TypeOptions quantization: Truncate | Round  (unbiased: +/- Inf) | Round  (unbiased: Even Values)
      mask TypeOptions overflow: Wrap | Saturate | Flag as error
      mask TypeOptions multiplier_implementation: behavioral HDL | standard core | embedded multiplier core
  cmac3 : Subsystem  Tag=cmac  AncestorBlock=casper_library_correlator/cmac  mask(cmac){acc_len=256, n_bits_a=8, bin_pt_a=7, n_bits_b=8, bin_pt_b=7, quantization=Truncate, overflow=Wrap, mult_latency=4, add_latency=3, in_latency=0, conv_latency=0, multiplier_implementation=embedded multiplier core}
      mask prompts: acc_len "Number of Accumulations"; n_bits_a "Number of bits 'a'"; bin_pt_a "Binary point 'a'"; n_bits_b "Number of bits 'b'"; bin_pt_b "Binary point 'b'"; quantization "Quantisation"; mult_latency "Multiplier Latency"; add_latency "Adder Latency"; in_latency "Input Latency"; conv_latency "Convert Latency"; multiplier_implementation "Multiplier Implementation"
      mask help: A complex multiply-accumulate block. Full precision.
      mask init: same as s_b16a4x1kf/sys0/xeng/auto_tap/dual_pol_cmac/cmac
      mask TypeOptions quantization: Truncate | Round  (unbiased: +/- Inf) | Round  (unbiased: Even Values)
      mask TypeOptions overflow: Wrap | Saturate | Flag as error
      mask TypeOptions multiplier_implementation: behavioral HDL | standard core | embedded multiplier core
  acc_out : Outport
  valid_out : Outport  Port=2
  wires:
  Constant2/1 -> cmac/5(valid_in)
  Slice/1 -> cmac/1(a+bi)
  Slice1/1 -> cmac/2(c+di)
  Slice2/1 -> cmac/3(acc_in)
  Slice3/1 -> cmac1/1(a+bi)
  Slice4/1 -> cmac1/2(c+di)
  Slice5/1 -> cmac1/3(acc_in)
  Concat/1 -> acc_out/1
  valid_in/1 -> cmac3/5(valid_in)
  cmac/2(valid_out) -> Terminator/1
  Constant1/1 -> cmac1/5(valid_in)
  Slice6/1 -> cmac2/1(a+bi)
  Slice7/1 -> cmac2/2(c+di)
  Slice8/1 -> cmac2/3(acc_in)
  Constant4/1 -> cmac2/5(valid_in)
  Slice9/1 -> cmac3/1(a+bi)
  Slice10/1 -> cmac3/2(c+di)
  Slice11/1 -> cmac3/3(acc_in)
  sync/1 -> cmac/4(sync), cmac1/4(sync), cmac2/4(sync), cmac3/4(sync)
  cmac1/2(valid_out) -> Terminator1/1
  cmac2/2(valid_out) -> Terminator2/1
  cmac3/2(valid_out) -> valid_out/1
  cmac/1(acc_out) -> Concat/1
  cmac1/1(acc_out) -> Concat/2
  cmac2/1(acc_out) -> Concat/3
  cmac3/1(acc_out) -> Concat/4
  a1/1 -> Slice/1, Slice3/1, Slice6/1, Slice9/1
  a2/1 -> Slice1/1, Slice4/1, Slice7/1, Slice10/1
  acc_in/1 -> Slice11/1, Slice8/1, Slice5/1, Slice2/1

== system s_b16a4x1kf/sys1/xeng/baseline_tap4/delay ==
  din : Inport
  constant : xbsIndex_r4/Constant  const=1  gui_display_data_type=Fixed-point  arith_type=Boolean  n_bits=16  bin_pt=14  preci_type=Single  exp_width=8  frac_width=24  explicit_period=on  period=1  equ=P=C  opselect=C  inp2=PCIN>>17  opr=+  inp1=P  carry=CIN  dbl_ovrd=off  block_type=constant
  counter : xbsIndex_r4/Counter  cnt_type=Count Limited  cnt_to=DelayLen - bram_latency - 1  operation=Up  start_count=0  cnt_by_val=1  arith_type=Unsigned  n_bits=8  bin_pt=0  load_pin=off  rst=off  en=off  explicit_period=on  period=1  use_behavioral_HDL=on  implementation=Fabric  use_rpm=off  dbl_ovrd=off  block_type=counter
  d{1..6} (6 alike) : xbsIndex_r4/Delay  rst=off  infoeditControl=Selection of Reset will increase slice count due to use of real FFs and instead of SRLs  en=off  latency=1  reg_retiming=on  dbl_ovrd=off  block_type=delay
  ram : xbsIndex_r4/Single Port RAM  depth=256  initVector=0  distributed_mem=Block RAM  write_mode=Read Before Write  rst=off  init_reg=0  en=off  latency=1  optimize=Area  dbl_ovrd=off  block_type=spram
  dout : Outport
  wires:
  counter/1 -> ram/1
  din/1 -> ram/2
  constant/1 -> ram/3
  ram/1 -> d1/1
  d1/1 -> d2/1
  d2/1 -> d3/1
  d3/1 -> d4/1
  d4/1 -> d5/1
  d5/1 -> d6/1
  d6/1 -> dout/1
